simulink model "wheatstone_bridge"  (R2025b)
settings: Solver=VariableStepAuto  StartTime=0.0  StopTime=5  RelTol=1e-3
libraries: fl_lib x13, nesl_utility x3, ee_lib x1, simulink_extras x1

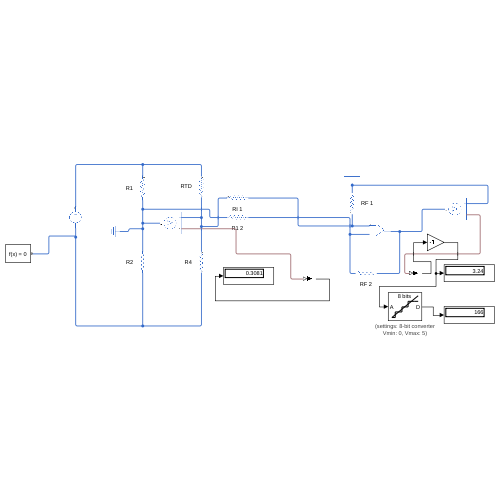
[thumbnail: Simulink's stored preview of the top-level diagram]
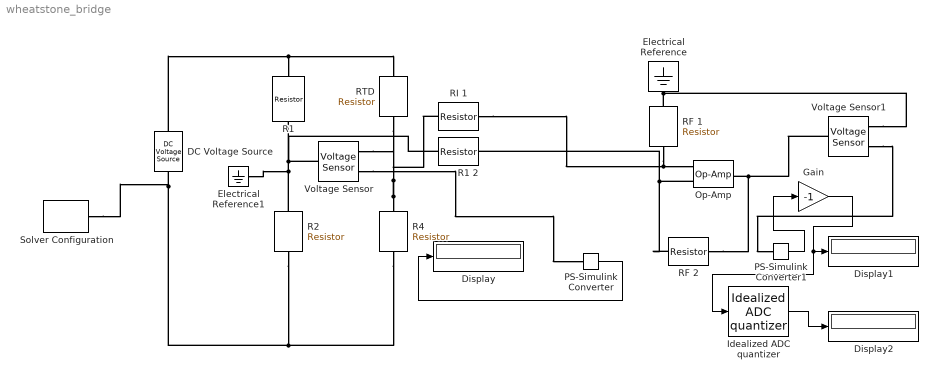
== system wheatstone_bridge ==
  DC Voltage Source : ee_lib/Additional Components/SPICE Sources/DC Voltage Source  DC=5 V
  Display : Display
  Display1 : Display
  Display2 : Display
  Electrical Reference : fl_lib/Electrical/Electrical Elements/Electrical Reference
  Electrical Reference1 : fl_lib/Electrical/Electrical Elements/Electrical Reference
  Gain : Gain  Gain=-1
  Idealized ADC quantizer : simulink_extras/Additional Discrete/Idealized ADC quantizer  NumberOfConverterBits=8  Vmin=0  Vmax=5  OutputDataType=int16  OutputNegativeValues=off
  Op-Amp : fl_lib/Electrical/Electrical Elements/Op-Amp  outI_specify=off  outI_priority=None  outI=0 A  outI_nominal_specify=off  outI_nominal_value=1  outI_nominal_unit=A
  PS-Simulink Converter : nesl_utility/PS-Simulink Converter  PhysicalDomain=network_engine_domain  SubClassName=ps_output  LeftPortType=input  RightPortType=output  PseudoPeriodic=off  Frequencies=[]  VectorFormat=inherit  Unit=inherit  AffineConversion=off
  PS-Simulink Converter1 : nesl_utility/PS-Simulink Converter  PhysicalDomain=network_engine_domain  SubClassName=ps_output  LeftPortType=input  RightPortType=output  PseudoPeriodic=off  Frequencies=[]  VectorFormat=inherit  Unit=inherit  AffineConversion=off
  R1 : fl_lib/Electrical/Electrical Elements/Resistor  R=1128.3 Ohm  i_specify=off  i_priority=None  i=0 A  i_nominal_specify=off  i_nominal_value=1  i_nominal_unit=A  v_specify=off  v_priority=None  v=0 V  v_nominal_specify=off  v_nominal_value=1  v_nominal_unit=V
  R1 2 : fl_lib/Electrical/Electrical Elements/Resistor  R=1000 kOhm  i_specify=off  i_priority=None  i=0 A  i_nominal_specify=off  i_nominal_value=1  i_nominal_unit=A  v_specify=off  v_priority=None  v=0 V  v_nominal_specify=off  v_nominal_value=1  v_nominal_unit=V
  R2 : fl_lib/Electrical/Electrical Elements/Resistor  R=1128.3 Ohm  i_specify=off  i_priority=None  i=0 A  i_nominal_specify=off  i_nominal_value=1  i_nominal_unit=A  v_specify=off  v_priority=None  v=0 V  v_nominal_specify=off  v_nominal_value=1  v_nominal_unit=V
  R4 : fl_lib/Electrical/Electrical Elements/Resistor  R=1128.3 Ohm  i_specify=off  i_priority=None  i=0 A  i_nominal_specify=off  i_nominal_value=1  i_nominal_unit=A  v_specify=off  v_priority=None  v=0 V  v_nominal_specify=off  v_nominal_value=1  v_nominal_unit=V
  RF 1 : fl_lib/Electrical/Electrical Elements/Resistor  R=10517.459 kOhm  i_specify=off  i_priority=None  i=0 A  i_nominal_specify=off  i_nominal_value=1  i_nominal_unit=A  v_specify=off  v_priority=None  v=0 V  v_nominal_specify=off  v_nominal_value=1  v_nominal_unit=V
  RF 2 : fl_lib/Electrical/Electrical Elements/Resistor  R=10517.459 kOhm  i_specify=off  i_priority=None  i=0 A  i_nominal_specify=off  i_nominal_value=1  i_nominal_unit=A  v_specify=off  v_priority=None  v=0 V  v_nominal_specify=off  v_nominal_value=1  v_nominal_unit=V
  RI 1 : fl_lib/Electrical/Electrical Elements/Resistor  R=1000 kOhm  i_specify=off  i_priority=None  i=0 A  i_nominal_specify=off  i_nominal_value=1  i_nominal_unit=A  v_specify=off  v_priority=None  v=0 V  v_nominal_specify=off  v_nominal_value=1  v_nominal_unit=V
  RTD : fl_lib/Electrical/Electrical Elements/Resistor  R=1445.5 Ohm  i_specify=off  i_priority=None  i=0 A  i_nominal_specify=off  i_nominal_value=1  i_nominal_unit=A  v_specify=off  v_priority=None  v=0 V  v_nominal_specify=off  v_nominal_value=1  v_nominal_unit=V
  Solver Configuration : nesl_utility/Solver Configuration  PhysicalDomain=network_engine_domain  SubClassName=solver  LeftPortType=input  RightPortType=generic  Tones=[]  Harmonics=[]  SimulateNoise=off  Profile=off  UseLocalSampling=off  EnableSwitchedLinearOptims=on  FrequencyDomain=off  UseCCode=off  RelTol=0.001  AbsTol=0.001  MinStep=1e-09  ToWorkspace=off  RevertToSquareIcSolve=off  NumHomotopyIterations=100  PhasorMode=off  PhasorModeNumHarmonics=1  ConsistencySolver=NEWTON_XTOL_AFTER_FTOL  IndexReductionMethod=DerivativeReplacement  DoDC=off  ResidualTolerance=1e-09  ConsistencyTolSource=GLOBAL  ConsistencyAbsTol=0.001  ConsistencyRelTol=0.001  ConsistencyTolFactor=0.001  UseLocalSolver=off  LocalSolverChoice=NE_BACKWARD_EULER_ADVANCER  ResolveIndetEquations=on  FunctionEvalNumThread=1  LocalSolverSampleTime=0.001  DoFixedCost=off  MaxNonlinIter=3  MaxModeIter=2  ComputeImpulses=off  ImpulseIterations=2  LinearAlgebra=auto  LinearAlgebraNumThread=0  EquationFormulation=NE_TIME_EF  DelaysMemoryBudget=1024  AutomaticFiltering=on  FilteringTimeConstant=0.001  PartitionStorageMethod=AS_NEEDED  PartitionMemoryBudget=1024  PartitionMethod=ROBUST  MultibodyUseLocalSolver=off  MultibodyLocalSolverChoice=ODE1  MultibodyLocalSolverSampleTime=0.001
  Voltage Sensor : fl_lib/Electrical/Electrical Sensors/Voltage Sensor
  Voltage Sensor1 : fl_lib/Electrical/Electrical Sensors/Voltage Sensor
  wires:
  PS-Simulink Converter/1 -> Display/1
  PS-Simulink Converter1/1 -> Gain/1
  Idealized ADC quantizer/1 -> Display2/1
  Gain/1 -> Idealized ADC quantizer/1, Display1/1
  connections:
  R2/RConn1 -- R4/RConn1 -- Solver Configuration/RConn1 -- DC Voltage Source/RConn1
  R2/LConn1 -- Electrical Reference1/LConn1 -- R1 2/LConn1 -- R1/RConn1 -- Voltage Sensor/LConn1
  Voltage Sensor/RConn1 -- PS-Simulink Converter/LConn1
  DC Voltage Source/LConn1 -- RTD/LConn1 -- R1/LConn1
  R4/LConn1 -- RI 1/LConn1 -- RTD/RConn1 -- Voltage Sensor/RConn2
  RI 1/RConn1 -- RF 1/LConn1 -- Op-Amp/LConn1
  Op-Amp/LConn2 -- RF 2/LConn1 -- R1 2/RConn1
  RF 2/RConn1 -- Voltage Sensor1/LConn1 -- Op-Amp/RConn1
  Voltage Sensor1/RConn1 -- PS-Simulink Converter1/LConn1
  RF 1/RConn1 -- Voltage Sensor1/RConn2 -- Electrical Reference/LConn1
